simulink model "g1_centroidal_reference"  (R2025b)
settings: Solver=FixedStepDiscrete  StartTime=0.0  StopTime=4.8  FixedStep=0.002  RelTol=1e-3
settings Model: DataDictionary=g1_data.sldd  EnableAccessToBaseWorkspace=off  Creator=enoch  LastModifiedBy=enoch

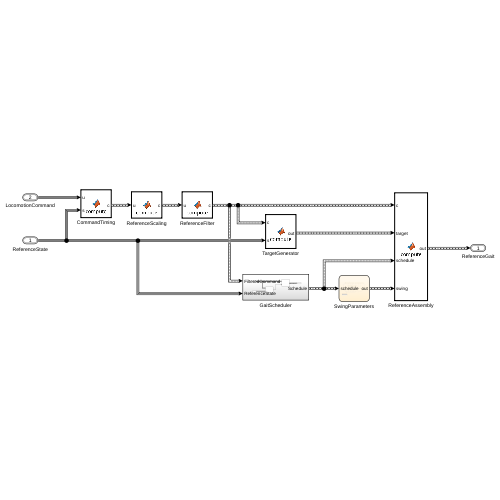
[thumbnail: Simulink's stored preview of the top-level diagram]
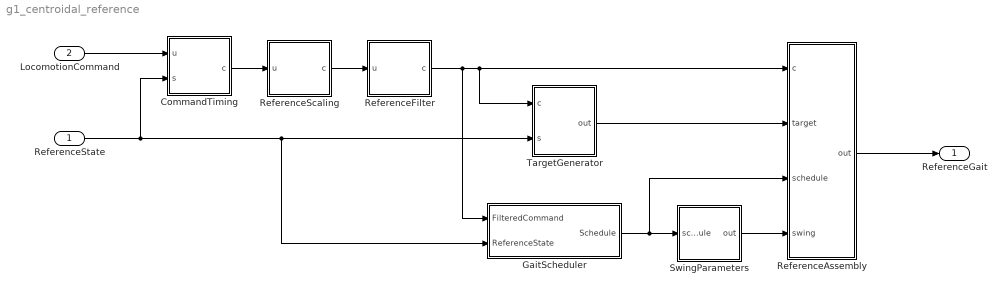
== system g1_centroidal_reference ==
  ReferenceState : Inport  OutDataTypeStr=Bus: ReferenceObservation  SampleTime=0.002
  LocomotionCommand : Inport  Port=2  OutDataTypeStr=Bus: LocomotionCommand  SampleTime=0.002
  CommandTiming : MATLAB Function  TreatAsAtomicUnit=on
  GaitScheduler : Subsystem  Description=GaitScheduler: SI command/WB58 -> complete raw mode schedule (s, mode0/1/2/3). Authoritative seven-state original selection guards, dwell0.2s, pruning, tiling, insertion and duplicate STANCE events. Sources: humanoid_nmpc/humanoid_common_mpc/src/gait/{GaitSchedule,GaitScheduleUpdater}.cpp and reference_manager/ProceduralMpcMotionManager.cpp. Updates only at real MPC requests.
  ReferenceAssembly : MATLAB Function  TreatAsAtomicUnit=on
  ReferenceFilter : MATLAB Function  TreatAsAtomicUnit=on
  ReferenceScaling : MATLAB Function  TreatAsAtomicUnit=on
  SwingParameters : Stateflow chart  TreatAsAtomicUnit=on
  TargetGenerator : MATLAB Function  TreatAsAtomicUnit=on
  ReferenceGait : Outport  OutDataTypeStr=Bus: ReferenceGait  BusOutputAsStruct=on
  wires:
  GaitScheduler/1(Schedule) -> ReferenceAssembly/3(schedule), SwingParameters/1(schedule)
  LocomotionCommand/1 -> CommandTiming/1(u)
  ReferenceState/1 -> GaitScheduler/2(ReferenceState), TargetGenerator/2(s), CommandTiming/2(s)
  CommandTiming/1(c) -> ReferenceScaling/1(u)
  ReferenceScaling/1(c) -> ReferenceFilter/1(u)
  ReferenceFilter/1(c) -> ReferenceAssembly/1(c), TargetGenerator/1(c), GaitScheduler/1(FilteredCommand)
  TargetGenerator/1(out) -> ReferenceAssembly/2(target)
  SwingParameters/1(out) -> ReferenceAssembly/4(swing)
  ReferenceAssembly/1(out) -> ReferenceGait/1

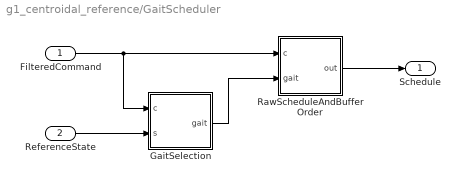
== system g1_centroidal_reference/GaitScheduler ==
  FilteredCommand : Inport  OutDataTypeStr=Bus: ProcessedCommand
  ReferenceState : Inport  Port=2  OutDataTypeStr=Bus: ReferenceObservation
  GaitSelection : Stateflow chart  TreatAsAtomicUnit=on
  RawScheduleAndBufferOrder : MATLAB Function  TreatAsAtomicUnit=on
  Schedule : Outport  OutDataTypeStr=Bus: GaitSchedule
  wires:
  GaitSelection/1(gait) -> RawScheduleAndBufferOrder/2(gait)
  ReferenceState/1 -> GaitSelection/2(s)
  FilteredCommand/1 -> RawScheduleAndBufferOrder/1(c), GaitSelection/1(c)
  RawScheduleAndBufferOrder/1(out) -> Schedule/1

== matlab function g1_centroidal_reference/CommandTiming ==
  data: u input Bus: LocomotionCommand; s input Bus: ReferenceObservation; c output Bus: ProcessedCommand
function c = compute(u, s)
%#codegen
% 命令发布时序：把物理观测 tick 转成规范时间，并决定是否发布新参考。
% u 为 LocomotionCommand；s 为包含 tick/session/epoch 的 ReferenceObservation。
c = processCommand(s, u);
end

function command = processCommand(observation, inputCommand)
% 物理控制周期为 2 ms；参考按 80 Hz 的截止时间发布。
% 重复 tick 只读取已有结果；session 或 epoch 改变时重新开始计时。
persistent session epoch nextSlot lastTick initialized

if isempty(initialized)
    initialized = false;
    session = uint64(0);
    epoch = uint64(0);
    nextSlot = uint64(0);
    lastTick = uint64(0);
end

reset = ~initialized || observation.session ~= session || observation.epoch ~= epoch;
time = double(observation.tick)*0.002;
assert(isfinite(observation.raw_backend_time) && ...
    abs(observation.raw_backend_time-time) <= 1e-12);

if reset
    session = observation.session;
    epoch = observation.epoch;
    nextSlot = uint64(0);
    initialized = true;
else
    assert(observation.tick >= lastTick, 'Control tick rollback requires a new epoch.');
end

% 使用首次到达截止时间的物理观测，不另建一套参考时钟。
request = reset || (observation.tick > lastTick && ...
    time+1e-12 >= double(nextSlot)/80);
if request
    nextSlot = nextSlot+uint64(1);
end
lastTick = observation.tick;

% values 顺序固定为：前向速度、侧向速度、绝对高度、偏航角速度。
command = struct('tick',observation.tick,'session',session,'epoch',epoch, ...
    'time',time,'request',request,'reset',reset, ...
    'values',[inputCommand.vx;inputCommand.vy;inputCommand.height;inputCommand.yaw_rate]);
end

== matlab function g1_centroidal_reference/ReferenceScaling ==
  data: u input Bus: ProcessedCommand; c output Bus: ProcessedCommand
function c = compute(u)
%#codegen
% 命令缩放：保持命令总线中的身份、时序和发布标志不变。
c = scaleCommand(u);
end

function command = scaleCommand(inputCommand)
% 四个通道依次为 vx、vy、绝对高度、偏航角速度。
% 只对两个平移速度通道缩放，不对高度增加偏置或限幅。
command = inputCommand;
command.values = inputCommand.values.*[2;1.2;1;1];
end

== matlab function g1_centroidal_reference/ReferenceFilter ==
  data: u input Bus: ProcessedCommand; c output Bus: ProcessedCommand
function c = compute(u)
%#codegen
% 命令低通滤波：仅在 request 为真时更新一次内部状态。
c = filterCommand(u);
end

function command = filterCommand(inputCommand)
% 一阶低通滤波，截止频率为 5 Hz，dt 取相邻参考发布时间之差。
persistent filteredValues lastUpdateTime
if isempty(filteredValues)
    filteredValues = zeros(4,1);
    lastUpdateTime = 0;
end

% 新 session/epoch 的首帧直接采用当前命令，避免沿用上一轮滤波状态。
if inputCommand.reset
    filteredValues = inputCommand.values;
    lastUpdateTime = inputCommand.time;
end

if inputCommand.request
    dt = inputCommand.time-lastUpdateTime;
    assert(dt >= 0);
    if dt ~= 0
        alpha = dt/(dt+1/(2*pi*5));
        filteredValues = alpha*inputCommand.values+(1-alpha)*filteredValues;
        lastUpdateTime = inputCommand.time;
    end
end

command = inputCommand;
command.values = filteredValues;
end

== matlab function g1_centroidal_reference/TargetGenerator ==
  data: c input Bus: ProcessedCommand; out output Bus: TargetTrajectories; s input Bus: ReferenceObservation
function out = compute(c, s)
%#codegen
% 目标轨迹生成：c 为滤波后的命令，s 为当前参考观测。
out = generateTargets(c, s);
end

function out = generateTargets(command, observation)
% 状态排列：位置 1:3，ZYX 欧拉角 4:6，关节角 7:29，
% 世界系线速度 30:32，ZYX 欧拉角导数 33:35，关节速度 36:58。
% active 是当前发布的轨迹；generated 是本次生成、供下一次发布的轨迹。
coder.cinclude('math.h');
persistent previousCommand targetBuffer initialized
if isempty(initialized)
    previousCommand = zeros(4,1);
    targetBuffer = emptyTarget();
    initialized = false;
end

% 首次发布只有一个节点：保留当前位姿和关节角，清零速度、俯仰和滚转。
if command.reset
    previousCommand = zeros(4,1);
    targetBuffer = emptyTarget();
    targetBuffer.active_count = uint32(1);
    targetBuffer.active_time(1) = command.time;
    initialState = observation.x;
    initialState(30:58) = 0;
    initialState(5:6) = 0;
    targetBuffer.active_state(:,1) = initialState;
    initialized = true;
end

if command.request
    % 先发布上一轮 generated，再计算下一轮；保留原有的一次发布延迟。
    % reset 首帧继续使用上面的单节点轨迹。
    if targetBuffer.active_count ~= uint32(1) || ~command.reset
        targetBuffer.active_count = uint32(3);
        targetBuffer.active_time = targetBuffer.generated_time;
        targetBuffer.active_state = targetBuffer.generated_state;
        targetBuffer.active_input = targetBuffer.generated_input;
    end

    % 第二级命令平滑，系数 0.8；与前一块的 5 Hz 滤波分别保留。
    previousCommand = previousCommand*0.8+command.values*(1-0.8);

    % 用当前观测的偏航角，将机体系水平速度命令旋转到世界系。
    yaw = observation.x(4);
    % 仿真生成代码继续调用 C 标准数学库，保持既有三角函数调用路径。
    if coder.target('MATLAB')
        cosYaw = cos(yaw);
        sinYaw = sin(yaw);
    else
        cosYaw = 0.0;
        sinYaw = 0.0;
        cosYaw = coder.ceval('cos',yaw);
        sinYaw = coder.ceval('sin',yaw);
    end
    worldCommand = previousCommand;
    worldCommand(1) = cosYaw*previousCommand(1)-sinYaw*previousCommand(2);
    worldCommand(2) = sinYaw*previousCommand(1)+cosYaw*previousCommand(2);

    % 三个目标节点覆盖 1.1 s；前 70% 用当前速度与命令速度的平均值积分。
    basePose = observation.x(1:6);
    basePose(3) = worldCommand(3);
    basePose(5:6) = 0;
    horizon = 1.2;
    firstDuration = 0.7*horizon;
    secondDuration = horizon-firstDuration;
    % 此处使用 ZYX 偏航角导数；完整运动学参考随后转为质心动量参考。
    averageVelocity = [(observation.x(30)+worldCommand(1))/2; ...
        (observation.x(31)+worldCommand(2))/2; ...
        (observation.x(33)+worldCommand(4))/2];
    middlePose = integratePlanarPose(basePose,averageVelocity,firstDuration);
    finalPose = integratePlanarPose(middlePose, ...
        [worldCommand(1);worldCommand(2);worldCommand(4)],secondDuration);

    % 23 个 MPC 关节的标称角度（rad）；节点速度顺序与完整状态一致。
    nominalJointAngles = [-0.05;0;0;0.1;-0.05;0;-0.05;0;0;0.1;-0.05;0;zeros(11,1)];
    desiredVelocity = [worldCommand(1);worldCommand(2);0;worldCommand(4);0;0;zeros(23,1)];
    targetBuffer.generated_time = [command.time;command.time+firstDuration;command.time+horizon];
    targetBuffer.generated_state = [[basePose;nominalJointAngles;desiredVelocity], ...
        [middlePose;nominalJointAngles;desiredVelocity],[finalPose;nominalJointAngles;desiredVelocity]];
end
out = targetBuffer;
end

function pose = integratePlanarPose(pose,velocity,dt)
% 只积分世界系 x/y 位置及偏航角，保持高度，并将俯仰、滚转目标置零。
pose(1) = pose(1)+velocity(1)*dt;
pose(2) = pose(2)+velocity(2)*dt;
pose(4) = pose(4)+velocity(3)*dt;
pose(5:6) = 0;
end

function target = emptyTarget()
% 固定容量总线：最多 3 个节点，每个节点含 58 维状态、35 维输入。
% 当前目标生成器不填充输入参考，因此输入数组保持初始化的零值。
target = struct('active_count',uint32(0), ...
    'active_time',zeros(3,1),'active_state',zeros(58,3),'active_input',zeros(35,3), ...
    'generated_time',zeros(3,1),'generated_state',zeros(58,3),'generated_input',zeros(35,3));
end

== matlab function g1_centroidal_reference/ReferenceAssembly ==
  data: c input Bus: ProcessedCommand; out output Bus: ReferenceGait; target input Bus: TargetTrajectories; schedule input Bus: GaitSchedule; swing input Bus: SwingReference
function out = compute(c, target, schedule, swing)
%#codegen
% 汇总参考总线：此处只组装字段，不更新滤波、目标轨迹或步态状态。
out = packReference(c, target, schedule, swing);
end

function out = packReference(command, target, schedule, swing)
% 四部分依次为命令及发布身份、目标轨迹、接触时间表、摆腿参数。
out = struct('command',command,'target',target,'schedule',schedule,'swing',swing);
end

== stateflow chart g1_centroidal_reference/SwingParameters ==
  state STANCE_INITIAL
    en, du: out=makeSwingReference(schedule); out.left_support=true; out.right_support=true;
  state STANCE_AFTER_RIGHT_SWING
    en, du: out=makeSwingReference(schedule); out.left_support=true; out.right_support=true;
  state FLY
    en, du: out=makeSwingReference(schedule); out.left_support=false; out.right_support=false;
  state LF_SUPPORT_RIGHT_SWING
    en, du: out=makeSwingReference(schedule); out.left_support=true; out.right_support=false;
  state RF_SUPPORT_LEFT_SWING
    en, du: out=makeSwingReference(schedule); out.left_support=false; out.right_support=true;
  (default) -> STANCE_INITIAL
  RF_SUPPORT_LEFT_SWING -> STANCE_INITIAL [order 1] : [schedule.current_mode == uint8(3)]
  STANCE_AFTER_RIGHT_SWING -> RF_SUPPORT_LEFT_SWING [order 1] : [schedule.current_mode == uint8(1)]
  STANCE_INITIAL -> RF_SUPPORT_LEFT_SWING [order 2] : [schedule.current_mode == uint8(1)]
  STANCE_INITIAL -> FLY [order 3] : [schedule.current_mode == uint8(0)]
  FLY -> STANCE_INITIAL [order 1] : [schedule.current_mode == uint8(3)]
  STANCE_INITIAL -> LF_SUPPORT_RIGHT_SWING [order 1] : [schedule.current_mode == uint8(2)]
  STANCE_AFTER_RIGHT_SWING -> FLY [order 3] : [schedule.current_mode == uint8(0)]
  STANCE_AFTER_RIGHT_SWING -> LF_SUPPORT_RIGHT_SWING [order 2] : [schedule.current_mode == uint8(2)]
  LF_SUPPORT_RIGHT_SWING -> STANCE_AFTER_RIGHT_SWING [order 1] : [schedule.current_mode == uint8(3)]
  FLY -> RF_SUPPORT_LEFT_SWING [order 3] : [schedule.current_mode == uint8(1)]
  RF_SUPPORT_LEFT_SWING -> FLY [order 3] : [schedule.current_mode == uint8(0)]
  FLY -> LF_SUPPORT_RIGHT_SWING [order 2] : [schedule.current_mode == uint8(2)]
  LF_SUPPORT_RIGHT_SWING -> FLY [order 3] : [schedule.current_mode == uint8(0)]
  LF_SUPPORT_RIGHT_SWING -> RF_SUPPORT_LEFT_SWING [order 2] : [schedule.current_mode == uint8(1)]
  RF_SUPPORT_LEFT_SWING -> LF_SUPPORT_RIGHT_SWING [order 2] : [schedule.current_mode == uint8(2)]
  data: gaitSchedule function_input; reference function_output; schedule input Bus: GaitSchedule; out output Bus: SwingReference
  function reference = makeSwingReference(gaitSchedule):
    | function reference = makeSwingReference(gaitSchedule)
    | % 摆腿配置：向 MPC 侧既有样条生成器提供参数和当前支撑状态。
    | % 接触模式：0=腾空，1=右脚支撑，2=左脚支撑，3=双脚支撑。
    | mode = gaitSchedule.current_mode;
    | 
    | % parameters 顺序与 SwingTrajectoryPlanner::Config 的消费约定一致：
    | % 1 离地竖直速度（m/s），2 落地竖直速度（m/s），3 摆腿高度（m），
    | % 4 落地高度偏置（m），5 短摆腿时长缩放阈值（s），
    | % 6 离地邻域速度系数，7 落地邻域速度系数，8 中点值系数。
    | % 第 2 项保留原来的负零，避免无意改变参数的二进制表示。
    | reference = struct('parameters',[.05;-0.0;.08;-.001;.4;-.15;.3;0], ...
    |     'terrain_height',0.0, ...
    |     'left_support',mode == uint8(2) || mode == uint8(3), ...
    |     'right_support',mode == uint8(1) || mode == uint8(3));
    | end

== stateflow chart g1_centroidal_reference/GaitScheduler/GaitSelection ==
  state RUN
    en, du: gait = uint8(6);
  state STANCE
    en: gait = uint8(0); lastChange = 0;
    du: gait = uint8(0);
  state TROT
    en, du: gait = uint8(5);
  state SLOW_TROT
    en, du: gait = uint8(4);
  state SLOWER_TROT
    en, du: gait = uint8(3);
  state WALK
    en, du: gait = uint8(2);
  state SLOW_WALK
    en, du: gait = uint8(1);
  RUN -> TROT [order 2] : [c.request && ~c.reset && c.time > lastChange + 0.2 && ~shouldIncreaseGait(c.values,s.x,uint8(6)) && shouldDecreaseGait(c.values,s.x,uint8(6))]/{lastChange = c.time;}
  TROT -> RUN [order 2] : [c.request && ~c.reset && c.time > lastChange + 0.2 && shouldIncreaseGait(c.values,s.x,uint8(5))]/{lastChange = c.time;}
  RUN -> STANCE [order 1] : [c.reset]/{lastChange = 0;}
  (default) -> STANCE
  TROT -> STANCE [order 1] : [c.reset]/{lastChange = 0;}
  SLOW_TROT -> STANCE [order 1] : [c.reset]/{lastChange = 0;}
  SLOWER_TROT -> STANCE [order 1] : [c.reset]/{lastChange = 0;}
  WALK -> STANCE [order 1] : [c.reset]/{lastChange = 0;}
  SLOW_WALK -> STANCE [order 3] : [c.request && ~c.reset && c.time > lastChange + 0.2 && ~shouldIncreaseGait(c.values,s.x,uint8(1)) && shouldDecreaseGait(c.values,s.x,uint8(1))]/{lastChange = c.time;}
  SLOW_WALK -> STANCE [order 1] : [c.reset]/{lastChange = 0;}
  STANCE -> SLOW_WALK : [c.request && ~c.reset && c.time > lastChange + 0.2 && shouldIncreaseGait(c.values,s.x,uint8(0))]/{lastChange = c.time;}
  SLOW_TROT -> TROT [order 2] : [c.request && ~c.reset && c.time > lastChange + 0.2 && shouldIncreaseGait(c.values,s.x,uint8(4))]/{lastChange = c.time;}
  SLOW_TROT -> SLOWER_TROT [order 3] : [c.request && ~c.reset && c.time > lastChange + 0.2 && ~shouldIncreaseGait(c.values,s.x,uint8(4)) && shouldDecreaseGait(c.values,s.x,uint8(4))]/{lastChange = c.time;}
  SLOWER_TROT -> WALK [order 3] : [c.request && ~c.reset && c.time > lastChange + 0.2 && ~shouldIncreaseGait(c.values,s.x,uint8(3)) && shouldDecreaseGait(c.values,s.x,uint8(3))]/{lastChange = c.time;}
  WALK -> SLOW_WALK [order 3] : [c.request && ~c.reset && c.time > lastChange + 0.2 && ~shouldIncreaseGait(c.values,s.x,uint8(2)) && shouldDecreaseGait(c.values,s.x,uint8(2))]/{lastChange = c.time;}
  TROT -> SLOW_TROT [order 3] : [c.request && ~c.reset && c.time > lastChange + 0.2 && ~shouldIncreaseGait(c.values,s.x,uint8(5)) && shouldDecreaseGait(c.values,s.x,uint8(5))]/{lastChange = c.time;}
  SLOWER_TROT -> SLOW_TROT [order 2] : [c.request && ~c.reset && c.time > lastChange + 0.2 && shouldIncreaseGait(c.values,s.x,uint8(3))]/{lastChange = c.time;}
  WALK -> SLOWER_TROT [order 2] : [c.request && ~c.reset && c.time > lastChange + 0.2 && shouldIncreaseGait(c.values,s.x,uint8(2))]/{lastChange = c.time;}
  SLOW_WALK -> WALK [order 2] : [c.request && ~c.reset && c.time > lastChange + 0.2 && shouldIncreaseGait(c.values,s.x,uint8(1))]/{lastChange = c.time;}
  data: commandValues function_input; state function_input; gaitIndex function_input; result function_output; commandValues function_input; state function_input; gaitIndex function_input; result function_output; gaitIndex function_input; parameters function_output; c input Bus: ProcessedCommand; s input Bus: ReferenceObservation; gait output uint8; lastChange local double; GaitTransitionParameters parameter double size=[7 6]
  function result = shouldIncreaseGait(commandValues, state, gaitIndex):
    | function result = shouldIncreaseGait(commandValues, state, gaitIndex)
    | % 升档判据：命令超过当前步态上界，且观测运动满足带误差余量的阈值。
    | % commandValues=[vx;vy;height;yaw_rate]；state(30:31) 为世界系水平速度，
    | % state(33) 为偏航欧拉角导数。速度单位为 m/s，角速度单位为 rad/s。
    | parameters = gaitParameters(gaitIndex);
    | result = (abs(commandValues(1)) > parameters(2) || ...
    |     abs(commandValues(2)) > parameters(2) || abs(commandValues(4)) > parameters(4)) && ...
    |     (abs(state(30)) > parameters(2)-parameters(5) || ...
    |     abs(state(31)) > parameters(2)-parameters(5) || ...
    |     abs(state(33)) > parameters(4)-parameters(6));
    | end
  function result = shouldDecreaseGait(commandValues, state, gaitIndex):
    | function result = shouldDecreaseGait(commandValues, state, gaitIndex)
    | % 降档判据：命令低于当前步态下界，且满足带误差余量的低速条件。
    | % 最后一项沿用命令偏航角速度，不在本次整理中替换为观测角速度。
    | parameters = gaitParameters(gaitIndex);
    | result = (abs(commandValues(1)) < parameters(1) && ...
    |     abs(commandValues(2)) < parameters(1) && abs(commandValues(4)) < parameters(3)) && ...
    |     (abs(state(30)) < parameters(1)+parameters(5) && ...
    |     abs(state(31)) < parameters(1)+parameters(5) && ...
    |     abs(commandValues(4)) < parameters(3)+parameters(6));
    | end
  function parameters = gaitParameters(gaitIndex):
    | function parameters = gaitParameters(gaitIndex)
    | % 从数据字典参数读取步态切换阈值；步态编号 0:6 对应参数表第 1:7 行。
    | % 编号：0站立、1慢走、2行走、3更慢小跑、4慢小跑、5小跑、6跑步。
    | % 列：1线速度下界、2线速度上界、3偏航角速度下界、4偏航角速度上界，
    | %     5线速度误差余量、6偏航角速度误差余量。
    | configurations = GaitTransitionParameters;
    | assert(gaitIndex <= 6);
    | parameters = configurations(double(gaitIndex)+1,:);
    | end

== matlab function g1_centroidal_reference/GaitScheduler/RawScheduleAndBufferOrder ==
  data: c input Bus: ProcessedCommand; out output Bus: GaitSchedule; gait input uint8
function out = compute(c, gait)
%#codegen
% 接触时间表维护：c 提供参考发布时间，gait 为状态机选出的步态编号。
out = updateGaitSchedule(c, gait);
end

function out = updateGaitSchedule(command, gait)
% 接触模式：0腾空、1右脚支撑、2左脚支撑、3双脚支撑。
% eventCount 个切换时刻对应 eventCount+1 个模式；数组容量固定为 64/65。
persistent eventTimes modes eventCount templateGait previousGait heldSchedule
if isempty(eventCount)
    eventCount = uint32(1);
    eventTimes = zeros(64,1);
    eventTimes(1) = 0.5;
    modes = uint8(3)*ones(65,1,'uint8');
    templateGait = uint8(0);
    previousGait = uint8(0);
    heldSchedule = emptySchedule();
end

% 新 session/epoch 从站立时间表开始，清除上一轮的步态模板和输出缓存。
if command.reset
    eventCount = uint32(1);
    eventTimes(:) = 0;
    eventTimes(1) = .5;
    modes(:) = uint8(3);
    templateGait = uint8(0);
    previousGait = uint8(0);
    heldSchedule = emptySchedule();
end

if command.request
    time = command.time;
    horizonEnd = time+1.2;
    horizonLength = horizonEnd-time;

    % 先用旧模板扩展窗口，并冻结本次输出；后面的步态切换作用于后续发布。
    [eventTimes,modes,eventCount] = trimAndExtendSchedule(eventTimes,modes,eventCount, ...
        templateGait,time-horizonLength,horizonEnd+horizonLength);
    heldSchedule.event_count = eventCount;
    heldSchedule.event_times = eventTimes;
    heldSchedule.modes = modes;
    heldSchedule.gait_index = gait;
    heldSchedule.current_mode = modeAt(eventTimes,modes,eventCount,time);
    heldSchedule.terminal_time = eventTimes(double(eventCount))+1;

    if gait ~= previousGait
        [eventTimes,modes,eventCount] = trimAndExtendSchedule(eventTimes,modes,eventCount, ...
            templateGait,time,horizonEnd+horizonLength);
        % 保留原浮点表达式的计算顺序，避免改变混合事件边界。
        earliestSwitch = .7*horizonEnd+.3*time;
        eventIndex = 1;
        while eventIndex <= double(eventCount) && eventTimes(eventIndex) <= earliestSwitch
            eventIndex = eventIndex+1;
        end

        if eventIndex > double(eventCount)
            switchTime = horizonEnd;
        elseif modeAt(eventTimes,modes,eventCount,eventTimes(eventIndex)) == uint8(2)
            assert(eventIndex > 1);
            switchTime = eventTimes(eventIndex-1);
        else
            switchTime = eventTimes(eventIndex);
        end

        % 截断切换点后的旧事件，再接上新模板；过渡站立时长保持为零。
        templateGait = gait;
        eventIndex = 1;
        while eventIndex <= double(eventCount) && eventTimes(eventIndex) < switchTime
            eventIndex = eventIndex+1;
        end
        eventCount = uint32(eventIndex-1);
        [eventTimes,modes,eventCount] = appendGaitCycles(eventTimes,modes,eventCount, ...
            templateGait,switchTime,1.5*horizonLength);
        previousGait = gait;
    end
end
out = heldSchedule;
end

function [eventTimes,modes,eventCount] = trimAndExtendSchedule( ...
    eventTimes,modes,eventCount,gait,windowStart,windowEnd)
% 裁剪窗口左侧历史事件时保留边界所需事件，并沿用首模式为站立的规则。
eventIndex = 1;
while eventIndex <= double(eventCount) && eventTimes(eventIndex) < windowStart
    eventIndex = eventIndex+1;
end
if eventIndex > 1
    removeCount = eventIndex-2;
    keepCount = double(eventCount)-removeCount;
    eventTimes(1:keepCount) = eventTimes(removeCount+1:double(eventCount));
    modes(1:keepCount+1) = modes(removeCount+1:double(eventCount)+1);
    eventCount = uint32(keepCount);
    modes(1) = uint8(3);
end

% 末尾事件先取下，再由模板扩展函数重新写入，保持原事件拼接顺序。
assert(eventCount > 0);
startTime = eventTimes(double(eventCount));
eventCount = eventCount-uint32(1);
[eventTimes,modes,eventCount] = appendGaitCycles( ...
    eventTimes,modes,eventCount,gait,startTime,windowEnd);
end

function [eventTimes,modes,eventCount] = appendGaitCycles( ...
    eventTimes,modes,eventCount,gait,startTime,endTime)
% 按完整步态周期追加，直至覆盖结束时间；保留重复的站立事件。
[phaseTimes,phaseModes,phaseCount] = gaitTemplate(gait);
if eventCount > 0
    assert(startTime > eventTimes(double(eventCount)));
end
eventCount = eventCount+uint32(1);
assert(eventCount <= 64);
eventTimes(double(eventCount)) = startTime;
while eventTimes(double(eventCount)) < endTime
    for phaseIndex = 1:phaseCount
        modes(double(eventCount)+1) = phaseModes(phaseIndex);
        duration = phaseTimes(phaseIndex+1)-phaseTimes(phaseIndex);
        eventCount = eventCount+uint32(1);
        assert(eventCount <= 64);
        eventTimes(double(eventCount)) = eventTimes(double(eventCount)-1)+duration;
    end
end
modes(double(eventCount)+1) = uint8(3);

% 只清空未使用容量，不合并或删除有效事件及模式。
eventTimes(double(eventCount)+1:64) = 0;
modes(double(eventCount)+2:65) = uint8(0);
end

function [times,modes,phaseCount] = gaitTemplate(gait)
% 相位时间单位为秒；编号对应 GaitSelection 的七个步态状态。
times = zeros(5,1);
modes = zeros(4,1,'uint8');
phaseCount = 1;
if gait == 0
    % 站立。
    times(2) = .5;
    modes(1) = uint8(3);
elseif gait == 1
    % 慢走：左支撑、双支撑、右支撑、双支撑。
    times = [0;.65;.85;1.5;1.7];
    modes = uint8([2;3;1;3]);
    phaseCount = 4;
elseif gait == 2
    % 行走。
    times = [0;.6;.7;1.3;1.4];
    modes = uint8([2;3;1;3]);
    phaseCount = 4;
elseif gait == 3
    % 更慢小跑：左右支撑交替。
    times(1:3) = [0;.6;1.2];
    modes(1:2) = uint8([2;1]);
    phaseCount = 2;
elseif gait == 4
    % 慢小跑。
    times(1:3) = [0;.55;1.1];
    modes(1:2) = uint8([2;1]);
    phaseCount = 2;
elseif gait == 5
    % 小跑。
    times(1:3) = [0;.5;1];
    modes(1:2) = uint8([2;1]);
    phaseCount = 2;
else
    % 跑步：左右支撑之间插入腾空相位，保留原来的兜底分支。
    times = [0;.3;.4;.7;.8];
    modes = uint8([2;0;1;0]);
    phaseCount = 4;
end
end

function mode = modeAt(eventTimes,modes,eventCount,time)
% 只越过严格早于查询时间的事件；恰好位于边界时沿用前一段模式。
eventIndex = 1;
while eventIndex <= double(eventCount) && eventTimes(eventIndex) < time
    eventIndex = eventIndex+1;
end
mode = modes(eventIndex);
end

function schedule = emptySchedule()
% terminal_time 是窗口外供消费端裁剪的标记，不是额外的实际切换事件。
schedule = struct('event_count',uint32(0),'event_times',zeros(64,1), ...
    'modes',zeros(65,1,'uint8'),'gait_index',uint8(0), ...
    'current_mode',uint8(3),'terminal_time',0.0);
end
